simulink library "Yaw_Actuation_Lib"  (R2025a)
settings: Solver=ode45  StartTime=0.0  StopTime=10.0  RelTol=1e-3  EnableMultiTasking=on
undefined symbols (not defined in the file): WT_Params
libraries: Yaw_Ideal_Actuator_Lib x4, Yaw_Ideal_Motor_Lib x4, Yaw_Motor_Lib x4
Description:
  | Copyright 2009-2025 The MathWorks, Inc. MathWorks, Inc.
settings Model: Creator=smiller  LastModifiedBy=smiller
settings SolverCC: AlgebraicLoopSolver=TrustRegion
settings DataIOCC: LimitDataPoints=on  SaveFormat=Array  SignalLoggingSaveFormat=ModelDataLogs  ReturnWorkspaceOutputs=off
settings OptimizationCC: ReuseModelBlockBuffer=off  ExpressionDepthLimit=2147483647.0  LifeSpan=inf
settings DebuggingCC: UnderspecifiedInitializationDetection=Classic  MergeDetectMultiDrivingBlocksExec=none  SolverPrmCheckMsg=warning  FcnCallInpInsideContextMsg=warning  UnconnectedInputMsg=warning  UnconnectedOutputMsg=warning  UnconnectedLineMsg=warning  AllowSymbolicDim=off  StateNameClashWarn=warning  PregeneratedLibrarySubsystemCodeDiagnostic=none  SFUnexpectedBacktrackingDiag=warning  SFNoUnconditionalDefaultTransitionDiag=warning  SFExecutionAtInitializationDiag=none  ArithmeticOperatorsInVariantConditions=warning
settings HardwareCC: ProdBitPerPointer=32.0  ProdBitPerSizeT=32.0  ProdBitPerPtrDiffT=32.0  ProdLargestAtomicFloat=None  ProdIntDivRoundTo=Undefined  ProdEndianess=Unspecified  ProdWordSize=32.0  ProdHWDeviceType=32-bit Generic
settings ModelReferenceCC: EnableRefExpFcnMdlSchedulingChecks=on  PropagateSignalLabelsOutOfModel=off
settings SFSimCC: SimUseLocalCustomCode=off  CustomCodeUndefinedFunction=UseInterfaceOnly
settings RTWCC: RTWUseLocalCustomCode=off  GPUComputeCapability=3.5  DLArmComputeVersion=19.05
settings CodeAppCC: StateflowObjectComments=on
settings GRTTargetCC: TargetLangStandard=C89/C90 (ANSI)  CombineOutputUpdateFcns=off  GRTInterface=on
settings ConfigComp: CovMetricSettings=dw  CovSaveCumulativeToWorkspaceVar=on  CovSaveSingleToWorkspaceVar=on  CovExternalEMLEnable=off  CovSFcnEnable=off

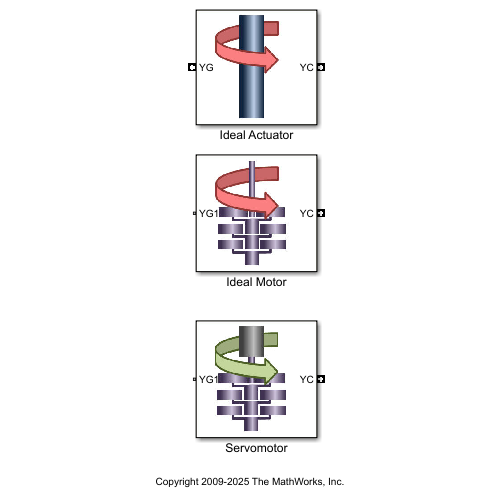
[thumbnail: Simulink's stored preview of the top-level diagram]
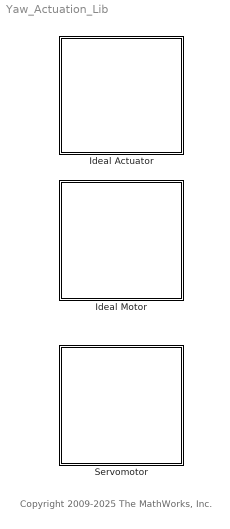
== system Yaw_Actuation_Lib ==
  note: Copyright 2009-2025 The MathWorks, Inc.
  Ideal Actuator : Subsystem
      mask Display: image('Yaw_Ideal_Actuation_IMAGE.jpg');
  Ideal Motor : Subsystem
      mask Display: image('Yaw_Ideal_Motors_IMAGE.jpg');
  Servomotor : Subsystem
      mask Display: image('Yaw_Servomotors_IMAGE.jpg');

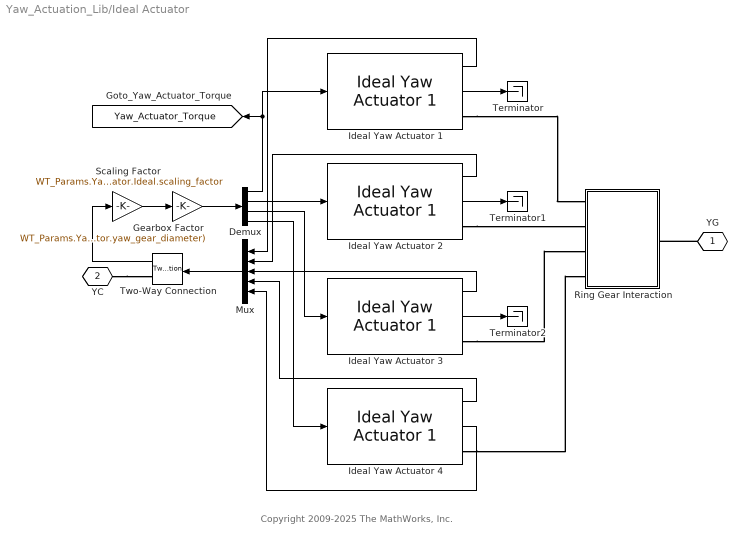
== system Yaw_Actuation_Lib/Ideal Actuator ==
  note: Copyright 2009-2025 The MathWorks, Inc.
  Demux : Demux
  Gearbox Factor : Gain  Gain=WT_Params.Yaw_Actuator.p_gear_rato_step_1*WT_Params.Yaw_Actuator.p_gear_rato_step_2*WT_Params.Yaw_Actuator.p_gear_rato_step_3*WT_Params.Yaw_Actuator.p_gear_rato_step_4*(WT_Params.Yaw_Actuator.yaw_ring_diameter/WT_Params.Yaw_Actuator.yaw_gear_diameter)
  Ideal Yaw Actuator {1..4} (4 alike) : Yaw_Ideal_Actuator_Lib/Ideal Yaw Actuator 1  SystemSampleTime=-1  VariantActivationTime=update diagram  EmptyChoice=off  PassThrough=off  PassThroughVariantControl=(default)  EmptyChoiceVariantControl=(default)  AllowFlexibleInterface=on  Latency=0  AutoFrameSizeCalculation=off
  Mux : Mux  Inputs=5
  Ring Gear Interaction : Subsystem
  Scaling Factor : Gain  Gain=WT_Params.Yaw_Actuator.Ideal.scaling_factor
  Terminator : Terminator
  Terminator1 : Terminator
  Terminator2 : Terminator
  Two-Way Connection : TwoWayConnection
  YG : PMIOPort  Tag=PMCPort  Side=Left
  YC : PMIOPort  Tag=PMCPort  Port=2  Side=Right
  tag scope: Yaw_Actuator_Torque=global
  wires:
  Scaling Factor/1 -> Gearbox Factor/1
  Ideal Yaw Actuator 4/1 -> Mux/4
  Ideal Yaw Actuator 3/1 -> Mux/3
  Ideal Yaw Actuator 2/1 -> Mux/2
  Demux/4 -> Ideal Yaw Actuator 4/1
  Demux/3 -> Ideal Yaw Actuator 3/1
  Demux/2 -> Ideal Yaw Actuator 2/1
  Ideal Yaw Actuator 4/2 -> Mux/5
  Ideal Yaw Actuator 3/2 -> Terminator2/1
  Ideal Yaw Actuator 2/2 -> Terminator1/1
  Ideal Yaw Actuator 1/2 -> Terminator/1
  Demux/1 -> [Yaw_Actuator_Torque], Ideal Yaw Actuator 1/1
  Two-Way Connection/1 -> Scaling Factor/1
  Ideal Yaw Actuator 1/1 -> Mux/1
  Gearbox Factor/1 -> Demux/1
  Mux/1 -> Two-Way Connection/1
  connections:
  Ideal Yaw Actuator 4/RConn1 -- Ring Gear Interaction/LConn4
  Ideal Yaw Actuator 3/RConn1 -- Ring Gear Interaction/LConn3
  Ideal Yaw Actuator 2/RConn1 -- Ring Gear Interaction/LConn2
  Ideal Yaw Actuator 1/RConn1 -- Ring Gear Interaction/LConn1
  YG/RConn1 -- Ring Gear Interaction/RConn1
  YC/RConn1 -- Two-Way Connection/RConn1

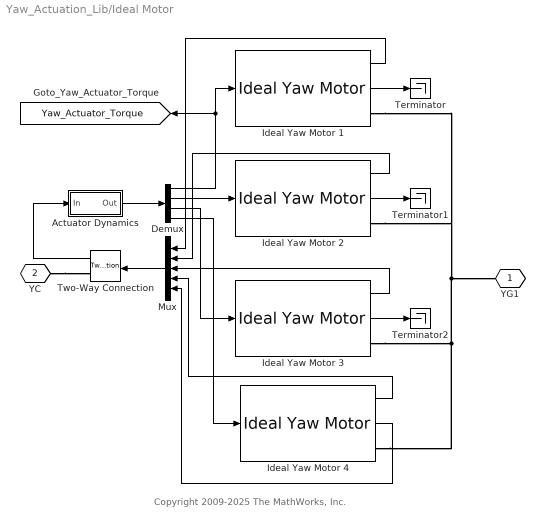
== system Yaw_Actuation_Lib/Ideal Motor ==
  note: Copyright 2009-2025 The MathWorks, Inc.
  Actuator Dynamics : Subsystem  mask(First-order lag supporting vector signals){b=WT_Params.Yaw_Actuator.ideal_actuator_time_constant, x_initial=0}
      mask prompts: b "Filter time constant"; x_initial "Initial output"
      mask help: Models a lag of the form 1/(b*s+1) where s is the Laplace operator.
  Demux : Demux
  Ideal Yaw Motor {1..4} (4 alike) : Yaw_Ideal_Motor_Lib/Ideal Yaw Motor  SystemSampleTime=-1  VariantActivationTime=update diagram  EmptyChoice=off  PassThrough=off  PassThroughVariantControl=(default)  EmptyChoiceVariantControl=(default)  AllowFlexibleInterface=on  Latency=0  AutoFrameSizeCalculation=off
  Mux : Mux  Inputs=5
  Terminator : Terminator
  Terminator1 : Terminator
  Terminator2 : Terminator
  Two-Way Connection : TwoWayConnection
  YG1 : PMIOPort  Tag=PMCPort  Side=Left
  YC : PMIOPort  Tag=PMCPort  Port=2  Side=Right
  tag scope: Yaw_Actuator_Torque=global
  wires:
  Ideal Yaw Motor 4/2 -> Mux/5
  Ideal Yaw Motor 4/1 -> Mux/4
  Ideal Yaw Motor 3/1 -> Mux/3
  Ideal Yaw Motor 2/1 -> Mux/2
  Ideal Yaw Motor 1/1 -> Mux/1
  Demux/4 -> Ideal Yaw Motor 4/1
  Demux/3 -> Ideal Yaw Motor 3/1
  Demux/2 -> Ideal Yaw Motor 2/1
  Demux/1 -> Ideal Yaw Motor 1/1, [Yaw_Actuator_Torque]
  Ideal Yaw Motor 3/2 -> Terminator2/1
  Ideal Yaw Motor 2/2 -> Terminator1/1
  Ideal Yaw Motor 1/2 -> Terminator/1
  Two-Way Connection/1 -> Actuator Dynamics/1(In)
  Mux/1 -> Two-Way Connection/1
  Actuator Dynamics/1(Out) -> Demux/1
  connections:
  YC/RConn1 -- Two-Way Connection/RConn1
  Ideal Yaw Motor 3/RConn1 -- Ideal Yaw Motor 2/RConn1 -- Ideal Yaw Motor 1/RConn1 -- YG1/RConn1 -- Ideal Yaw Motor 4/RConn1

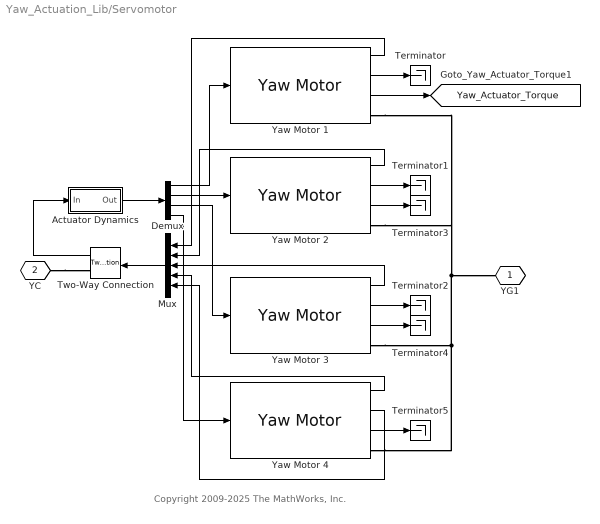
== system Yaw_Actuation_Lib/Servomotor ==
  note: Copyright 2009-2025 The MathWorks, Inc.
  Actuator Dynamics : Subsystem  mask(First-order lag supporting vector signals){b=WT_Params.Yaw_Actuator.ideal_actuator_time_constant, x_initial=0}
      mask prompts: b "Filter time constant"; x_initial "Initial output"
      mask help: Models a lag of the form 1/(b*s+1) where s is the Laplace operator.
  Demux : Demux
  Mux : Mux  Inputs=5
  Terminator{,1..5} (6 alike) : Terminator
  Two-Way Connection : TwoWayConnection
  Yaw Motor {1..4} (4 alike) : Yaw_Motor_Lib/Yaw Motor  SystemSampleTime=-1  VariantActivationTime=update diagram  EmptyChoice=off  PassThrough=off  PassThroughVariantControl=(default)  EmptyChoiceVariantControl=(default)  AllowFlexibleInterface=on  Latency=0  AutoFrameSizeCalculation=off
  YG1 : PMIOPort  Tag=PMCPort  Side=Left
  YC : PMIOPort  Tag=PMCPort  Port=2  Side=Right
  tag scope: Yaw_Actuator_Torque=global
  wires:
  Yaw Motor 4/3 -> Terminator5/1
  Yaw Motor 3/3 -> Terminator4/1
  Yaw Motor 2/3 -> Terminator3/1
  Yaw Motor 1/3 -> [Yaw_Actuator_Torque]
  Actuator Dynamics/1(Out) -> Demux/1
  Mux/1 -> Two-Way Connection/1
  Two-Way Connection/1 -> Actuator Dynamics/1(In)
  Yaw Motor 1/2 -> Terminator/1
  Yaw Motor 2/2 -> Terminator1/1
  Yaw Motor 3/2 -> Terminator2/1
  Demux/1 -> Yaw Motor 1/1
  Demux/2 -> Yaw Motor 2/1
  Demux/3 -> Yaw Motor 3/1
  Demux/4 -> Yaw Motor 4/1
  Yaw Motor 1/1 -> Mux/1
  Yaw Motor 2/1 -> Mux/2
  Yaw Motor 3/1 -> Mux/3
  Yaw Motor 4/1 -> Mux/4
  Yaw Motor 4/2 -> Mux/5
  connections:
  Yaw Motor 4/RConn1 -- YG1/RConn1 -- Yaw Motor 1/RConn1 -- Yaw Motor 2/RConn1 -- Yaw Motor 3/RConn1
  YC/RConn1 -- Two-Way Connection/RConn1

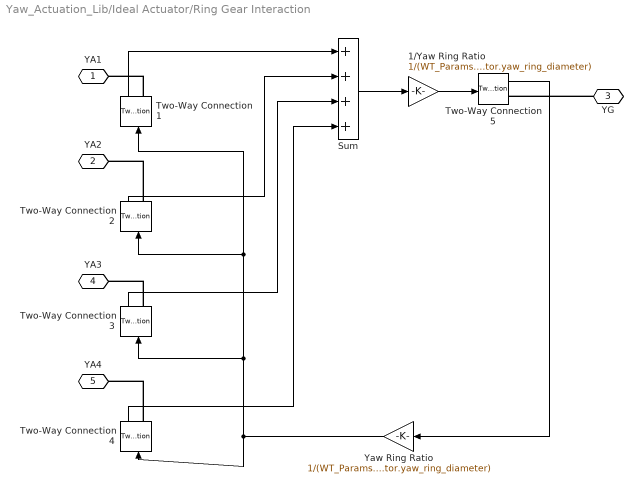
== system Yaw_Actuation_Lib/Ideal Actuator/Ring Gear Interaction ==
  1/Yaw Ring Ratio : Gain  Gain=1/(WT_Params.Yaw_Actuator.yaw_gear_diameter/WT_Params.Yaw_Actuator.yaw_ring_diameter)
  Sum : Sum  Inputs=++++
  Two-Way Connection{1..5} (5 alike) : TwoWayConnection
  Yaw Ring Ratio : Gain  Gain=1/(WT_Params.Yaw_Actuator.yaw_gear_diameter/WT_Params.Yaw_Actuator.yaw_ring_diameter)
  YA1 : PMIOPort  Side=Left
  YA2 : PMIOPort  Port=2  Side=Left
  YG : PMIOPort  Port=3  Side=Right
  YA3 : PMIOPort  Port=4  Side=Left
  YA4 : PMIOPort  Port=5  Side=Left
  wires:
  Yaw Ring Ratio/1 -> Two-Way Connection1/1, Two-Way Connection2/1, Two-Way Connection3/1, Two-Way Connection4/1
  Two-Way Connection4/1 -> Sum/4
  Sum/1 -> 1/Yaw Ring Ratio/1
  Two-Way Connection5/1 -> Yaw Ring Ratio/1
  Two-Way Connection3/1 -> Sum/3
  Two-Way Connection2/1 -> Sum/2
  Two-Way Connection1/1 -> Sum/1
  1/Yaw Ring Ratio/1 -> Two-Way Connection5/1
  connections:
  YG/RConn1 -- Two-Way Connection5/RConn1
  Two-Way Connection4/RConn1 -- YA4/RConn1
  Two-Way Connection3/RConn1 -- YA3/RConn1
  Two-Way Connection2/RConn1 -- YA2/RConn1
  Two-Way Connection1/RConn1 -- YA1/RConn1

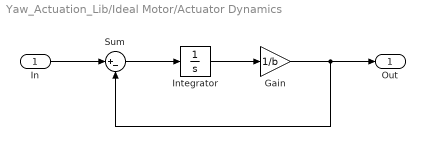
== system Yaw_Actuation_Lib/Ideal Motor/Actuator Dynamics ==
  In : Inport
  Gain : Gain  Gain=1/b
  Integrator : Integrator  InitialCondition=x_initial
  Sum : Sum  Inputs=|+-  InputSameDT=on  SaturateOnIntegerOverflow=on  OutDataTypeStr=Inherit: Same as first input
  Out : Outport  VectorParamsAs1DForOutWhenUnconnected=off
  wires:
  Gain/1 -> Out/1, Sum/2
  Integrator/1 -> Gain/1
  In/1 -> Sum/1
  Sum/1 -> Integrator/1

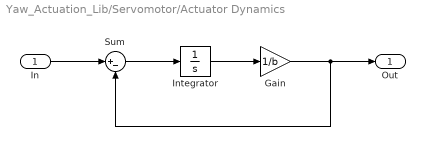
== system Yaw_Actuation_Lib/Servomotor/Actuator Dynamics ==
  In : Inport
  Gain : Gain  Gain=1/b
  Integrator : Integrator  InitialCondition=x_initial
  Sum : Sum  Inputs=|+-  InputSameDT=on  SaturateOnIntegerOverflow=on  OutDataTypeStr=Inherit: Same as first input
  Out : Outport  VectorParamsAs1DForOutWhenUnconnected=off
  wires:
  Sum/1 -> Integrator/1
  In/1 -> Sum/1
  Integrator/1 -> Gain/1
  Gain/1 -> Sum/2, Out/1
